simulink model "fixedWingPathFollowing"  (R2021b)
settings: Solver=FixedStepAuto  StartTime=0.0  StopTime=300  FixedStep=0.01  RelTol=1e-3
libraries: uavalgslib x4, robotcorelib x2, uavutilslib x2
settings Model: DataDictionary=fixedWingPathFollowingData.sldd  EnableAccessToBaseWorkspace=off  PacingRate=10  Creator=The MathWorks, Inc.  LastModifiedBy=Jihoon Lee
settings SolverCC: AlgebraicLoopSolver=TrustRegion  DecoupledContinuousIntegration=on
settings DataIOCC: ReturnWorkspaceOutputs=off
settings DebuggingCC: SFMachineParentedDataDiag=warning  ArithmeticOperatorsInVariantConditions=warning
settings SFSimCC: SimUseLocalCustomCode=off  CustomCodeUndefinedFunction=UseInterfaceOnly
settings RTWCC: RTWUseLocalCustomCode=off

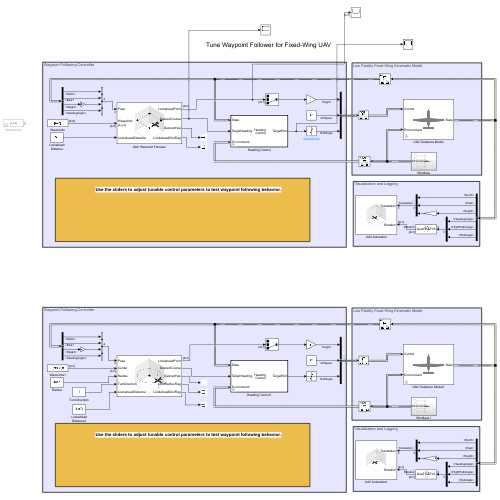
[thumbnail: Simulink's stored preview of the top-level diagram]
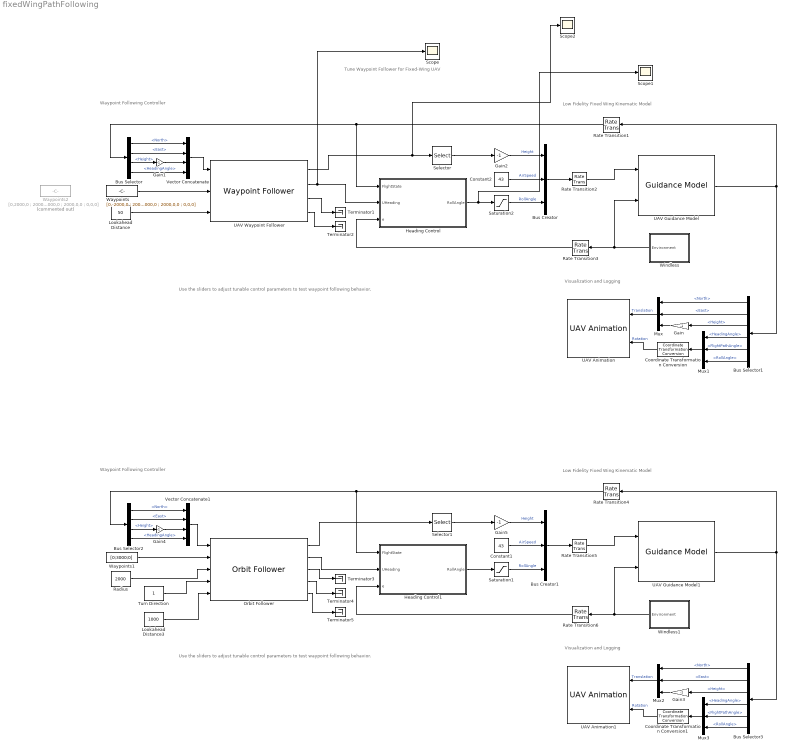
== system fixedWingPathFollowing ==
  note: Tune Waypoint Follower for Fixed-Wing UAV
  note: Use the sliders to adjust tunable control parameters to test waypoint following behavior.
  note: Visualization and Logging
  note: Low Fidelity Fixed Wing Kinematic Model
  note: Waypoint Following Controller
  note: Use the sliders to adjust tunable control parameters to test waypoint following behavior.
  note: Visualization and Logging
  note: Low Fidelity Fixed Wing Kinematic Model
  note: Waypoint Following Controller
  Bus Creator : BusCreator  Inputs=3  OutDataTypeStr=Bus: FixedWingControlBus  NonVirtualBus=on
  Bus Creator1 : BusCreator  Inputs=3  OutDataTypeStr=Bus: FixedWingControlBus  NonVirtualBus=on
  Bus Selector : BusSelector  OutputSignals=North,East,Height,HeadingAngle
  Bus Selector1 : BusSelector  OutputSignals=North,East,Height,HeadingAngle,FlightPathAngle,RollAngle
  Bus Selector2 : BusSelector  OutputSignals=North,East,Height,HeadingAngle
  Bus Selector3 : BusSelector  OutputSignals=North,East,Height,HeadingAngle,FlightPathAngle,RollAngle
  Constant1 : Constant  Value=43
  Constant2 : Constant  Value=43
  Coordinate Transformation Conversion : robotcorelib/Coordinate Transformation Conversion  InputRepresentation=Euler Angles  InputEulerSequence=ZYX  ShowTrVecInputPort=on  OutputRepresentation=Quaternion  OutputEulerSequence=ZYX  ShowTrVecOutputPort=on  SimulateUsing=Code generation
      settings: SourceProductBaseCode=NV,RO,RR,UV
  Coordinate Transformation Conversion1 : robotcorelib/Coordinate Transformation Conversion  InputRepresentation=Euler Angles  InputEulerSequence=ZYX  ShowTrVecInputPort=on  OutputRepresentation=Quaternion  OutputEulerSequence=ZYX  ShowTrVecOutputPort=on  SimulateUsing=Code generation
      settings: SourceProductBaseCode=NV,RO,RR,UV
  Gain{,1..5} (6 alike) : Gain  Gain=-1
  Heading Control : MATLAB Function  TreatAsAtomicUnit=on  mask(Fixed Wing Heading Controller){PHeadingAngle=1}
      mask prompts: PHeadingAngle "Heading Control Gain"
      mask help: P controller that regulates fixed wing UAV heading direction through controlling its roll angle. This controller requires that the plane is flying under coordinated flight condition.
  Heading Control1 : MATLAB Function  TreatAsAtomicUnit=on  mask(Fixed Wing Heading Controller){PHeadingAngle=0.39}
      mask prompts: PHeadingAngle "Heading Control Gain"
      mask help: P controller that regulates fixed wing UAV heading direction through controlling its roll angle. This controller requires that the plane is flying under coordinated flight condition.
  Lookahead Distance : Constant  Value=50
  Lookahead Distance3 : Constant  Value=1000
  Mux{,1..3} (4 alike) : Mux  Inputs=3
  Orbit Follower : uavalgslib/Orbit Follower  UAVType=fixed-wing  MinOrbitRadius=1  MinLookaheadDistance=0.1  ExternalReset=none  ShowCrossTrackErrorOutput=off  ShowNumTurnsOutput=off  SimulateUsing=Interpreted execution
      settings: SourceProductBaseCode=UV
  Radius : Constant  Value=2000
  Rate Transition{1,3..4,6} (4 alike) : RateTransition  OutPortSampleTime=0.01
  Rate Transition2 : RateTransition  OutPortSampleTime=0.1
  Rate Transition5 : RateTransition  OutPortSampleTime=0.1
  Saturation1 : Saturate  UpperLimit=20/180*pi  LowerLimit=-20/180*pi
  Saturation2 : Saturate  UpperLimit=20/180*pi  LowerLimit=-20/180*pi
  Scope : Scope
  Scope1 : Scope
  Scope2 : Scope
  Selector : Selector  InputPortWidth=3  IndexOptions=Index vector (dialog)  Indices=[3]  OutputSizes=1
  Selector1 : Selector  InputPortWidth=3  IndexOptions=Index vector (dialog)  Indices=[3]  OutputSizes=1
  Terminator{1..5} (5 alike) : Terminator
  Turn Direction : Constant
  UAV Animation : uavutilslib/UAV Animation  UAVType=FixedWing  UAVSize=50  InertialZDirection=Down  SampleTime=0.1
      settings: SourceProductBaseCode=UV
  UAV Animation1 : uavutilslib/UAV Animation  UAVType=FixedWing  UAVSize=50  InertialZDirection=Down  SampleTime=0.1
      settings: SourceProductBaseCode=UV
  UAV Guidance Model : uavalgslib/Guidance Model  ModelType=FixedWingGuidance  SpecifiedDataType=double  SimulateUsing=Code generation  InitialWorldPositionMultirotor=[0; 0; 0]  InitialWorldVelocityMultirotor=[0; 0; 0]  InitialEulerZYXMultirotor=[0; 0; 0]  InitialBodyAngularRateRPYMultirotor=[0; 0; 0]  InitialThrustMultirotor=0  InitialNorthFixedWing=0  InitialEastFixedWing=0  InitialHeightFixedWing=0  InitialAirSpeedFixedWing=43  InitialHeadingAngleFixedWing=pi/2  InitialFlightPathAngleFixedWing=0  InitialRollAngleFixedWing=0  InitialRollAngleRateFixedWing=0  PDRollMultirotor=[3402.97,116.67]  PDPitchMultirotor=[3402.97, 116.67]  PYawRateMultirotor=1950  PThrustMultirotor=3900  MassMultirotor=0.1  PHeightFixedWing=3.9  PHeadingAngleFixedWing=3.9  PFlightPathAngleFixedWing=39  PDRollFixedWing=[5.9414, 3.9]  PAirSpeedFixedWing=1  FlightPathAngleLimitsFixedWing=[-pi/6, pi/6]  StateBusName='FixedWingStateBus'  ControlBusName='FixedWingControlBus'  EnvironmentBusName='FixedWingEnvironmentBus'  DataType=double
      settings: SourceProductBaseCode=UV
  UAV Guidance Model1 : uavalgslib/Guidance Model  ModelType=FixedWingGuidance  SpecifiedDataType=double  SimulateUsing=Code generation  InitialWorldPositionMultirotor=[0; 0; 0]  InitialWorldVelocityMultirotor=[0; 0; 0]  InitialEulerZYXMultirotor=[0; 0; 0]  InitialBodyAngularRateRPYMultirotor=[0; 0; 0]  InitialThrustMultirotor=0  InitialNorthFixedWing=0  InitialEastFixedWing=0  InitialHeightFixedWing=0  InitialAirSpeedFixedWing=43  InitialHeadingAngleFixedWing=pi/2  InitialFlightPathAngleFixedWing=0  InitialRollAngleFixedWing=0  InitialRollAngleRateFixedWing=0  PDRollMultirotor=[3402.97,116.67]  PDPitchMultirotor=[3402.97, 116.67]  PYawRateMultirotor=1950  PThrustMultirotor=3900  MassMultirotor=0.1  PHeightFixedWing=3.9  PHeadingAngleFixedWing=3.9  PFlightPathAngleFixedWing=39  PDRollFixedWing=[5.9414, 3.9]  PAirSpeedFixedWing=1  FlightPathAngleLimitsFixedWing=[-pi/6, pi/6]  StateBusName='FixedWingStateBus'  ControlBusName='FixedWingControlBus'  EnvironmentBusName='FixedWingEnvironmentBus'  DataType=double
      settings: SourceProductBaseCode=UV
  UAV Waypoint Follower : uavalgslib/Waypoint Follower  UAVType=fixed-wing  StartFrom=first  TransitionRadiusSource=internal  TransitionRadius=100  MinLookaheadDistance=0.1  YawInput=off  ShowCrossTrackErrorOutput=off  ShowStatusOutput=off  SimulateUsing=Code generation
      settings: SourceProductBaseCode=UV
  Vector Concatenate : Concatenate  NumInputs=4
  Vector Concatenate1 : Concatenate  NumInputs=4
  Waypoints : Constant  Value=[0,-2000,0 ; 2000,2000,0 ; 2000,0,0 ; 0,0,0]  VectorParams1D=off
  Waypoints1 : Constant  Value=[0;3000;0]  VectorParams1D=off
  Waypoints2 : Constant  Commented=on  Value=[0,2000,0 ; 2000,2000,0 ; 2000,0,0 ; 0,0,0]  VectorParams1D=off
  Windless : Subsystem  VariantControl=NoWind
  Windless1 : Subsystem  VariantControl=NoWind
  wires:
  Constant2/1 -> Bus Creator/2  "AirSpeed"
  Gain2/1 -> Bus Creator/1  "Height"
  Bus Creator/1 -> Rate Transition2/1
  Bus Selector/1 -> Vector Concatenate/1  "<North>"
  Bus Selector/2 -> Vector Concatenate/2  "<East>"
  Saturation2/1 -> Bus Creator/3  "RollAngle"
  Rate Transition1/1 -> Heading Control/1(FlightState), Bus Selector/1
  Rate Transition2/1 -> UAV Guidance Model/1
  UAV Waypoint Follower/2 -> Scope/1, Heading Control/2(UHeading)
  UAV Waypoint Follower/1 -> Scope2/1, Selector/1
  Waypoints/1 -> UAV Waypoint Follower/2
  Vector Concatenate/1 -> UAV Waypoint Follower/1
  UAV Waypoint Follower/3 -> Terminator1/1
  Lookahead Distance/1 -> UAV Waypoint Follower/3
  Heading Control/1(RollAngle) -> Scope1/1, Saturation2/1
  Gain/1 -> Mux/3
  Bus Selector1/6 -> Mux1/3  "<RollAngle>"
  Bus Selector1/5 -> Mux1/2  "<FlightPathAngle>"
  Mux1/1 -> Coordinate Transformation Conversion/1
  Coordinate Transformation Conversion/1 -> UAV Animation/2  "Rotation"
  UAV Guidance Model/1 -> Bus Selector1/1, Rate Transition1/1
  Mux/1 -> UAV Animation/1  "Translation"
  Windless/1(Environment) -> UAV Guidance Model/2, Rate Transition3/1
  Bus Selector/4 -> Vector Concatenate/4  "<HeadingAngle>"
  Bus Selector/3 -> Gain1/1  "<Height>"
  Gain1/1 -> Vector Concatenate/3
  Selector/1 -> Gain2/1
  Rate Transition3/1 -> Heading Control/3(e)
  Bus Selector1/1 -> Mux/1  "<North>"
  Bus Selector1/2 -> Mux/2  "<East>"
  Bus Selector1/4 -> Mux1/1  "<HeadingAngle>"
  Bus Selector1/3 -> Gain/1  "<Height>"
  UAV Waypoint Follower/4 -> Terminator2/1
  Saturation1/1 -> Bus Creator1/3  "RollAngle"
  Orbit Follower/4 -> Terminator4/1
  Bus Selector3/4 -> Mux3/1  "<HeadingAngle>"
  Bus Selector3/3 -> Gain3/1  "<Height>"
  UAV Guidance Model1/1 -> Bus Selector3/1, Rate Transition4/1
  Bus Selector3/2 -> Mux2/2  "<East>"
  Bus Creator1/1 -> Rate Transition5/1
  Gain4/1 -> Vector Concatenate1/3
  Waypoints1/1 -> Orbit Follower/2
  Rate Transition6/1 -> Heading Control1/3(e)
  Orbit Follower/2 -> Heading Control1/2(UHeading)
  Bus Selector2/4 -> Vector Concatenate1/4  "<HeadingAngle>"
  Bus Selector3/1 -> Mux2/1  "<North>"
  Windless1/1(Environment) -> UAV Guidance Model1/2, Rate Transition6/1
  Bus Selector2/3 -> Gain4/1  "<Height>"
  Vector Concatenate1/1 -> Orbit Follower/1
  Selector1/1 -> Gain5/1
  Mux2/1 -> UAV Animation1/1  "Translation"
  Bus Selector3/6 -> Mux3/3  "<RollAngle>"
  Bus Selector2/1 -> Vector Concatenate1/1  "<North>"
  Bus Selector3/5 -> Mux3/2  "<FlightPathAngle>"
  Rate Transition5/1 -> UAV Guidance Model1/1
  Mux3/1 -> Coordinate Transformation Conversion1/1
  Coordinate Transformation Conversion1/1 -> UAV Animation1/2  "Rotation"
  Orbit Follower/1 -> Selector1/1
  Bus Selector2/2 -> Vector Concatenate1/2  "<East>"
  Gain3/1 -> Mux2/3
  Constant1/1 -> Bus Creator1/2  "AirSpeed"
  Radius/1 -> Orbit Follower/3
  Rate Transition4/1 -> Heading Control1/1(FlightState), Bus Selector2/1
  Orbit Follower/3 -> Terminator3/1
  Gain5/1 -> Bus Creator1/1  "Height"
  Heading Control1/1(RollAngle) -> Saturation1/1
  Turn Direction/1 -> Orbit Follower/4
  Lookahead Distance3/1 -> Orbit Follower/5
  Orbit Follower/5 -> Terminator5/1

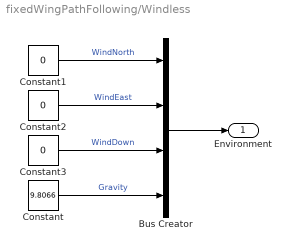
== system fixedWingPathFollowing/Windless ==
  Bus Creator : BusCreator  Inputs=4  OutDataTypeStr=Bus: FixedWingEnvironmentBus  NonVirtualBus=on
  Constant : Constant  Value=9.8066
  Constant1 : Constant  Value=0
  Constant2 : Constant  Value=0
  Constant3 : Constant  Value=0
  Environment : Outport  VectorParamsAs1DForOutWhenUnconnected=off
  wires:
  Constant2/1 -> Bus Creator/2  "WindEast"
  Constant3/1 -> Bus Creator/3  "WindDown"
  Constant1/1 -> Bus Creator/1  "WindNorth"
  Bus Creator/1 -> Environment/1
  Constant/1 -> Bus Creator/4  "Gravity"

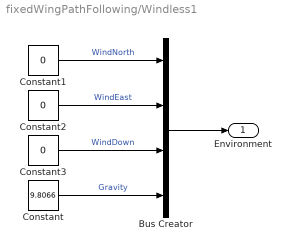
== system fixedWingPathFollowing/Windless1 ==
  Bus Creator : BusCreator  Inputs=4  OutDataTypeStr=Bus: FixedWingEnvironmentBus  NonVirtualBus=on
  Constant : Constant  Value=9.8066
  Constant1 : Constant  Value=0
  Constant2 : Constant  Value=0
  Constant3 : Constant  Value=0
  Environment : Outport  VectorParamsAs1DForOutWhenUnconnected=off
  wires:
  Constant2/1 -> Bus Creator/2  "WindEast"
  Constant3/1 -> Bus Creator/3  "WindDown"
  Constant1/1 -> Bus Creator/1  "WindNorth"
  Bus Creator/1 -> Environment/1
  Constant/1 -> Bus Creator/4  "Gravity"

== matlab function fixedWingPathFollowing/Heading Control1 ==
  data: FlightState input Bus: FixedWingStateBus; UHeading input; RollAngle output size=[1 1]; e input Bus: FixedWingEnvironmentBus; PHeadingAngle parameter
function RollAngle = fcn(FlightState, UHeading, e, PHeadingAngle)
    
    Va = FlightState.AirSpeed;
    HeadingAngle = FlightState.HeadingAngle;
    FlightPathAngle = FlightState.FlightPathAngle;
    
    YawAngle = HeadingAngle - asin((1/Va)*[e.WindNorth, e.WindEast]*[-sin(HeadingAngle); cos(HeadingAngle)]);
    b = [cos(HeadingAngle)*cos(FlightPathAngle), sin(HeadingAngle)*cos(FlightPathAngle), -sin(FlightPathAngle)]*[e.WindNorth; e.WindEast; e.WindDown];
    c = [e.WindNorth, e.WindEast, e.WindDown]*[e.WindNorth; e.WindEast; e.WindDown]- Va^2;
    Vg = -b+sqrt(b^2-c);
    
    RollAngle = atan2(PHeadingAngle*angdiff(HeadingAngle,UHeading)*Vg,e.Gravity*cos(HeadingAngle-YawAngle));

== matlab function fixedWingPathFollowing/Heading Control ==
  data: FlightState input Bus: FixedWingStateBus; UHeading input; RollAngle output size=[1 1]; e input Bus: FixedWingEnvironmentBus; PHeadingAngle parameter
function RollAngle = fcn(FlightState, UHeading, e, PHeadingAngle)
    
    Va = FlightState.AirSpeed;
    HeadingAngle = FlightState.HeadingAngle;
    FlightPathAngle = FlightState.FlightPathAngle;
    
    YawAngle = HeadingAngle - asin((1/Va)*[e.WindNorth, e.WindEast]*[-sin(HeadingAngle); cos(HeadingAngle)]);
    b = [cos(HeadingAngle)*cos(FlightPathAngle), sin(HeadingAngle)*cos(FlightPathAngle), -sin(FlightPathAngle)]*[e.WindNorth; e.WindEast; e.WindDown];
    c = [e.WindNorth, e.WindEast, e.WindDown]*[e.WindNorth; e.WindEast; e.WindDown]- Va^2;
    Vg = -b+sqrt(b^2-c);
    
    RollAngle = atan2(PHeadingAngle*angdiff(HeadingAngle,UHeading)*Vg,e.Gravity*cos(HeadingAngle-YawAngle));
